simulink model "sfDashboardBoiler"  (R2025b)
settings: Solver=ode45  StartTime=0.0  StopTime=1400  RelTol=1e-3  EnableMultiTasking=on
settings Model: PacingRate=50  ExtModeTrigMode=oneshot  ExtModeArmWhenConnect=off  ExtModeAutoUpdateStatusClock=off  Creator=The MathWorks, Inc.  LastModifiedBy=The MathWorks, Inc.
settings SolverCC: AlgebraicLoopSolver=TrustRegion  InsertRTBMode=Auto
settings DataIOCC: SaveFormat=Array  SaveOutput=off  SaveTime=off  ReturnWorkspaceOutputs=off  SignalLoggingName=sigsOut
settings OptimizationCC: BlockReduction=off  BooleanDataType=off  ReuseModelBlockBuffer=off  ExpressionDepthLimit=2147483647.0  InitFltsAndDblsToZero=on  LifeSpan=1  EfficientTunableParamExpr=on
settings DebuggingCC: SaveWithParameterizedLinksMsg=none  UnderspecifiedInitializationDetection=Classic  MergeDetectMultiDrivingBlocksExec=none  SignalResolutionControl=TryResolveAllWithWarning  MultiTaskDSMMsg=warning  MultiTaskCondExecSysMsg=none  ParameterPrecisionLossMsg=none  FcnCallInpInsideContextMsg=warning  UnconnectedInputMsg=warning  UnconnectedOutputMsg=warning  UnconnectedLineMsg=warning  StateNameClashWarn=warning  SFUnexpectedBacktrackingDiag=warning  SFNoUnconditionalDefaultTransitionDiag=warning  SFExecutionAtInitializationDiag=none  ArithmeticOperatorsInVariantConditions=warning
settings HardwareCC: ProdBitPerPointer=32.0  ProdBitPerSizeT=32.0  ProdBitPerPtrDiffT=32.0  ProdLargestAtomicFloat=None  ProdIntDivRoundTo=Undefined  ProdEndianess=Unspecified  ProdWordSize=32.0  ProdHWDeviceType=ASIC/FPGA  TargetUnknown=on  ProdEqTarget=off
settings ModelReferenceCC: EnableRefExpFcnMdlSchedulingChecks=on  PropagateSignalLabelsOutOfModel=off
settings SFSimCC: SFSimEcho=off  SimUseLocalCustomCode=off  SimParseCustomCode=off  CustomCodeUndefinedFunction=UseInterfaceOnly
settings RTWCC: SystemTargetFile=ert.tlc  GenCodeOnly=on  TemplateMakefile=ert_default_tmf  GenerateReport=on  RTWVerbose=off  RTWUseLocalCustomCode=off  IncludeHyperlinkInReport=on  LaunchReport=on  GPUComputeCapability=3.5  DLArmComputeVersion=19.05
settings CodeAppCC: IgnoreCustomStorageClasses=off  CustomSymbolStrType=$N$R$M  CustomSymbolStrModelFcn=$N  StateflowObjectComments=on  InternalIdentifier=Classic
settings ERTTargetCC: InlinedParameterPlacement=Hierarchical  ERTCustomFileTemplate=example_file_process.tlc  ConvertIfToSwitch=off  SuppressUnreachableDefaultCases=off  TargetFcnLib=ansi_tfl_tmw.mat  MultiwordLength=2048.0  GenerateSampleERTMain=on  SupportContinuousTime=on  SupportNonInlinedSFcns=on
settings ConfigComp: CovMetricSettings=dcmtr  CovSaveCumulativeToWorkspaceVar=on  CovSaveSingleToWorkspaceVar=on  CovExternalEMLEnable=off  CovSFcnEnable=off

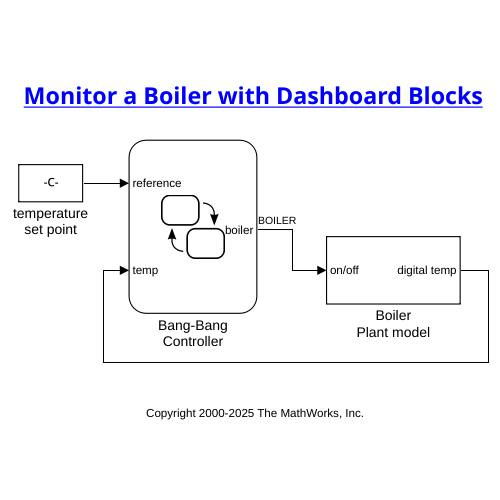
[thumbnail: Simulink's stored preview of the top-level diagram]
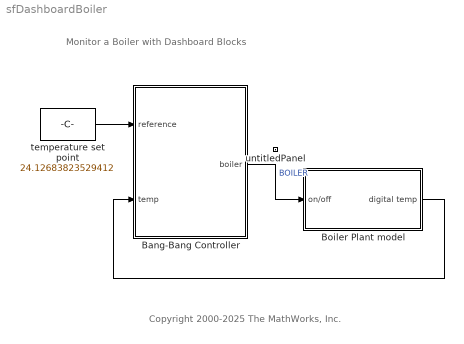
== system sfDashboardBoiler ==
  note: Copyright 2000-2025 The MathWorks, Inc.
  note: Monitor a Boiler with Dashboard Blocks
  Bang-Bang Controller : Stateflow chart  TreatAsAtomicUnit=on
  Boiler Plant model : Subsystem
  temperature set point : Constant  Value=24.12683823529412  OutDataTypeStr=Inherit: Inherit via back propagation
  untitledPanel : Subsystem  Tag=HiddenForWebPanel  IsWebBlockPanel=on
  wires:
  Bang-Bang Controller/1(boiler) -> Boiler Plant model/1(on/off)  "BOILER"
  temperature set point/1 -> Bang-Bang Controller/1(reference)
  Boiler Plant model/1(digital temp) -> Bang-Bang Controller/2(temp)

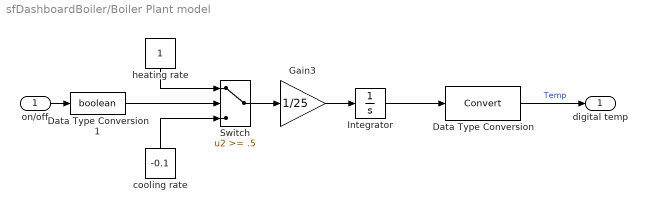
== system sfDashboardBoiler/Boiler Plant model ==
  on/off : Inport
  Data Type Conversion1 : DataTypeConversion  OutDataTypeStr=boolean
  Data Type Conversion : DataTypeConversion  SaturateOnIntegerOverflow=off  RndMeth=Floor
  Gain3 : Gain  Gain=1/25  SaturateOnIntegerOverflow=on  OutDataTypeStr=Inherit: Same as input  ParamDataTypeStr=Inherit: Same as input
  Integrator : Integrator  InitialCondition=15  ZeroCross=off
  Switch : Switch  Threshold=.5
  cooling rate : Constant  Value=-0.1
  heating rate : Constant
  digital temp : Outport
  wires:
  Gain3/1 -> Integrator/1
  cooling rate/1 -> Switch/3
  heating rate/1 -> Switch/1
  Switch/1 -> Gain3/1
  on/off/1 -> Data Type Conversion1/1
  Data Type Conversion1/1 -> Switch/2
  Integrator/1 -> Data Type Conversion/1
  Data Type Conversion/1 -> digital temp/1  "Temp"

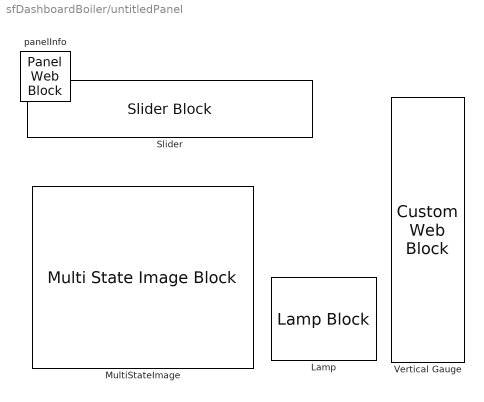
== system sfDashboardBoiler/untitledPanel ==
  Lamp : LampBlock  Tag=HiddenForWebPanel  PanelInfo="{\"height\":83,\"left\":266,\"panelId\":\"panelId-744c00eb-fe83-4cd3-9ee6-97a1be0f1a1a\",\"top\":241,\"type\":\"panelChild\",\"version\":\"2019b\",\"width\":105,\"zIndex\":1500008}"  LabelPosition=Hide  DefaultColor=[192.0, 192.0, 192.0]
  MultiStateImage : MultiStateImageBlock  Tag=HiddenForWebPanel  PanelInfo="{\"height\":182,\"left\":27,\"panelId\":\"panelId-744c00eb-fe83-4cd3-9ee6-97a1be0f1a1a\",\"top\":150,\"type\":\"panelChild\",\"version\":\"2019b\",\"width\":221,\"zIndex\":2000802}"  LabelPosition=Hide
  Slider : SliderBlock  Tag=HiddenForWebPanel  PanelInfo="{\"height\":57,\"left\":22,\"panelId\":\"panelId-744c00eb-fe83-4cd3-9ee6-97a1be0f1a1a\",\"top\":44,\"type\":\"panelChild\",\"version\":\"2019b\",\"width\":285,\"zIndex\":1500004}"  LabelPosition=Hide  ScaleMax=50
  Vertical Gauge : CustomWebBlock  Tag=HiddenForWebPanel  PanelInfo="{\"height\":265,\"left\":386,\"panelId\":\"panelId-744c00eb-fe83-4cd3-9ee6-97a1be0f1a1a\",\"top\":61,\"type\":\"panelChild\",\"version\":\"2019b\",\"width\":73,\"zIndex\":1500010}"  LabelPosition=Hide  ShowInitialText=on  Configuration="{\"components\":[{\"name\":\"LinearScaleComponent\",\"settings\":{\"bounds\":{\"max\":50,\"min\":0,\"tickInterval\":\"auto\"},\"labelColor\":[250,245,199],\"labelFont\":{\"font\":\"Arial\",\"fontSize\":12},\"labelOffset\":0.05,\"labelTransparency\":1,\"needleImage\":{\"size\":[21,75],\"src\":\"data:image\\/svg+xml;base64,PHN2ZyB4bWxucz0iaHR0cDovL3d3dy53My5vcmcvMjAwMC9zdmciIHhtbG5zOnhsaW5rPSJodHRwOi8vd3d3LnczLm9yZy8xOTk5L3hsaW5rIiB2aWV3Qm94PSIwIDAgMjEgNzUiPjxkZWZzPjxzdHlsZT4uY2xzLTF7ZmlsbDpub25lO30uY2xzLTJ7aXNvbGF0aW9uOmlzb2xhdGU7fS5jbHMtM3tjbGlwLXBhdGg6dXJsKCNjbGlwLXBhdGgpO30uY2xzLTR7b3BhY2l0eTowLjM7bWl4LWJsZW5kLW1vZGU6bXVsdGlwbHk7fS5jbHMtNXtmaWxsOiNlYjI2Mjk7fTwvc3R5bGU+PGNsaXBQYXRoIGlkPSJjbGlwLXBhdGgiIHRyYW5zZm9y ...(+1928 chars)\",\"srcOrientation\":\"horizontal\"},\"needleOffset\":[-0.01094391244870041,0],\"needleSize\":{\"height\":0.11960078534031414,\"width\":0.7589285714285714},\"position\":[0.015887605042016806,0.06986607142857143,0.8,0.9641544117647058],\"referencePoint\":\"auto\",\"scaleColorSize\":0.24,\"scaleColors\":[],\"scaleColorsSize\":0.2,\"scaleDirection\":\"BT\",\"tickColor\":[250,245,200],\"tickTransparency\":1,\"valueBarColor\":[23,89,176],\"valueBarSize\":0.23,\"valueBarTransparency\":1}},{\"name\":\"BackgroundImageComponent\",\"settings\":{\"image\":{\"size\":[101,380],\"src\":\"data:image\\/svg+xml;base64,PHN2ZyB4bWxucz0iaHR0cDovL3d3dy53My5vcmcvMjAwMC9zdmciIHZpZXdCb3g9IjAgMCAxMDEgMzgwIj48ZGVmcz48c3R5bGU+LmNscy0xe2ZpbGw6IzAwMmI0Mjt9LmNscy0ye2ZpbGw6IzQyNzA4Mjt9LmNscy0ze2ZpbGw6IzdjYTBiMjt9PC9zdHlsZT48L2RlZnM+PHRpdGxlPnZlcnRpY2FsX2dhdWdlX2JhY2tncm91bmRfMTwvdGl0bGU+PGcgaWQ9IkxheWVyXzIiIGRhdGEtbmFtZT0iTGF5ZXIgMiI+PGcgaWQ9IkxheWVyXzEtMiIgZGF0YS1uYW1lPSJMYXllciAxIj48cmVjdCBjbGFzcz0iY2xzLTEiIHg9IjExIiB5PSIxMSIgd2lkdGg9Ijc5IiBoZWlnaHQ9IjM1OCIvPjxwYXRoIGNsYXNzPSJjbHMtMiIgZD0iTTkzLDhIOFYzNzJIOTNaTTExLDM2OVYxMUg5MFYzNjlaIi8+PHBhdGggY2xhc3M9ImNscy0zIiBkPSJNMTAxLDBIMFYzODBIMTAxWk04LDM3MlY4SDkzVjM3MloiLz48L2c+PC9nPjwvc3ZnPg==\",\"srcOrientation\":\"vertical\"},\"position\":[0,0,1,1],\"scaleMode\":\"0\"}},{\"name\":\"ForegroundImageComponent\",\"settings\":{\"image\":{\"size\":[0,0],\"src\":\"default\",\"srcOrientation\":[]},\"isForeground\":1,\"position\":[0,0,1,1],\"scaleMode\":\"0\"}}],\"derived\":{\"blockParameters\":{\"ForegroundColor\":[0.9803921568627451,0.9607843137254902,0.7843137254901961],\"Limits\":{\"Max\":50,\"Min\":0,\"Ticks\":\"auto\"},\"ScaleColors\":[],\"ScaleDirection\":\"Clockwise\",\"ScaleMax\":50,\"ScaleMin\":0,\"TickInterval\":\"auto\",\"fixedAspectRatio\":\"on\"}},\"settings\":{\"BindingType\":\"signal\",\"backgroundColor\":[0,0,0],\"backgroundOffset\":0,\"backgroundOpacity\":1,\"fixedAspectRatio\":\"on\",\"orientation\":\"vertical\",\"showBackgroundColor\":0,\"version\":\"R2025a\"},\"type\":\"LinearGauge\"}"
  panelInfo : PanelWebBlock  Tag=HiddenForWebPanel  PanelInfo="{\"compacted\":false,\"height\":360,\"isActiveTab\":true,\"labels\":{\"label0580070817\":{\"left\":\"263\",\"settings\":{\"backgroundColor\":\"rgba(0, 0, 0, 0)\",\"bold\":true,\"font\":\"Arial\",\"fontColor\":\"black\",\"fontSize\":0.9,\"italicized\":false,\"underlined\":false},\"text\":\"Boiler On\\/Off\",\"top\":\"223\"},\"label4541398475\":{\"left\":\"32\",\"settings\":{\"backgroundColor\":\"rgba(0, 0, 0, 0)\",\"bold\":true,\"font\":\"Arial\",\"fontColor\":\"black\",\"fontSize\":0.9,\"italicized\":false,\"underlined\":false},\"text\":\"Boiler Activity - High\\/Normal\\/Off\",\"top\":\"127\"},\"label4741137272\":{\"left\":\"382\",\"settings\":{\"backgroundColor\":\"rgba(0, 0, 0, 0)\",\"bold\":true,\"font\":\"Arial\",\"fontColor\":\"black\",\"fontSize\":0.9,\"italicized\":false,\"underlined\":false},\"text\":\"Temperature\",\"top\":\"14\"},\"label7573753281\":{\"left\":\"382\",\"settings\":{\"backgroundColor\":\"rgba(0, 0, 0, 0)\",\"bold\":true,\"font\":\"Arial\",\"fontColor\":\"black\",\"fontSize\":0.9,\"italicized\":false,\"underlined\":false},\"text\":\"Output\",\"top\":\"37\"},\"label9201257219\":{\"left\":\"23\",\"settings\":{\"backgroundColor\":\"rgba(0, 0, 0, 0)\",\"bold\":true,\"font\":\"Arial\",\"fontColor\":\"black\",\"fontSize\":0.9,\"italicized\":false,\"underlined\":false},\"text\":\"Temperature Setpoint\",\"top\":\"17\"}},\"left\":599,\"name\":\"untitledPanel\",\"panelId\":\"panelId-744c00eb-fe83-4cd3-9ee6-97a1be0f1a1a\",\"tabIndex\":0,\"tabbedSetId\":\"tabbedSet1260466485\",\"top\":61,\"type\":\"panel\",\"version\":\"2019b\",\"visible\":true,\"width\":478,\"zIndex\":1500002}"  PanelSnapshot=<binary blob, 42932 chars, not shown>

== stateflow chart sfDashboardBoiler/Bang-Bang Controller ==
  settings: updateMethod=DISCRETE  sampleTime=1
  state Heater [group]
    state Off
      entry: turn_boiler(OFF)
    state On
      en: turn_boiler(ON)
      (history)
      state HIGH
      state NORM
      state b = warm() [function]
        (default) -> (junction 41) : {b = ~cold()}
      (default) -> HIGH
      HIGH -> NORM : [warm()]
    (default) -> Off
    On -> Off : after(20,sec)
    Off -> On : after(40,sec)
        | [cold()]
    NORM -> Off : [Heater.On.warm()]
  state turn_boiler(mode) [function]
    (default) -> (junction 32)
    (junction 32) -> (junction 33) [order 1] : [mode==ON]
    (junction 32) -> (junction 43) [order 2] : {color=RED}
    (junction 33) -> (junction 35) : {color=GREEN}
    (junction 43) -> (junction 34)
    (junction 35) -> (junction 34)
    (junction 34) -> (junction 36) : {LED=color;
        |  boiler=mode}
  state b = cold() [function]
    (default) -> (junction 39) : { b = temp<=reference}
  data: b function_output boolean; mode function_input int8; b function_output boolean; boiler output int8; color local int8; reference input fixdt(1,8,1,-15); GREEN constant int8 =2; OFF constant int8; ON constant int8 =1; RED constant int8 =1; temp input uint16; LED local int8
